simulink model "simulacaoPI"  (R2023b)
settings: Solver=VariableStepAuto  StartTime=0.0  StopTime=0.05  RelTol=1e-3
values from neighbouring files (symbols this model uses):
  Cc = 0.000143    [PI_boost.m]
  Ts = 5.0e-5    (= 5e-05)    [PI_boost.m]
  Vs = 30    [PI_boost.m]
libraries: spsSeriesRLCBranchLib x3, spsCurrentMeasurementLib x1, spsDiodeLib x1, spsDCVoltageSourceLib x1, spsGroundLib x1, spsMosfetLib x1, spsPWMGeneratorDCDCLib x1, spsVoltageMeasurementLib x1, sps_lib x1
settings Model: Creator=luisf  LastModifiedBy=luisf

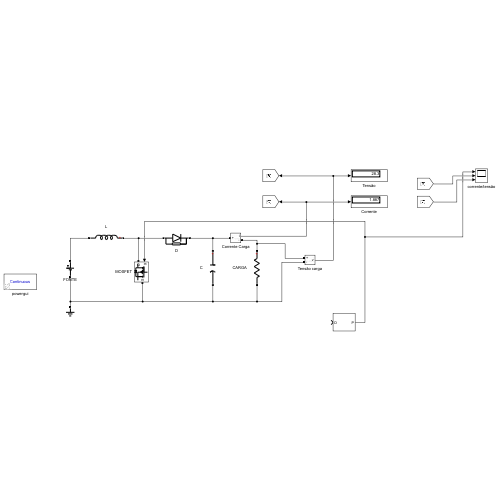
[thumbnail: Simulink's stored preview of the top-level diagram]
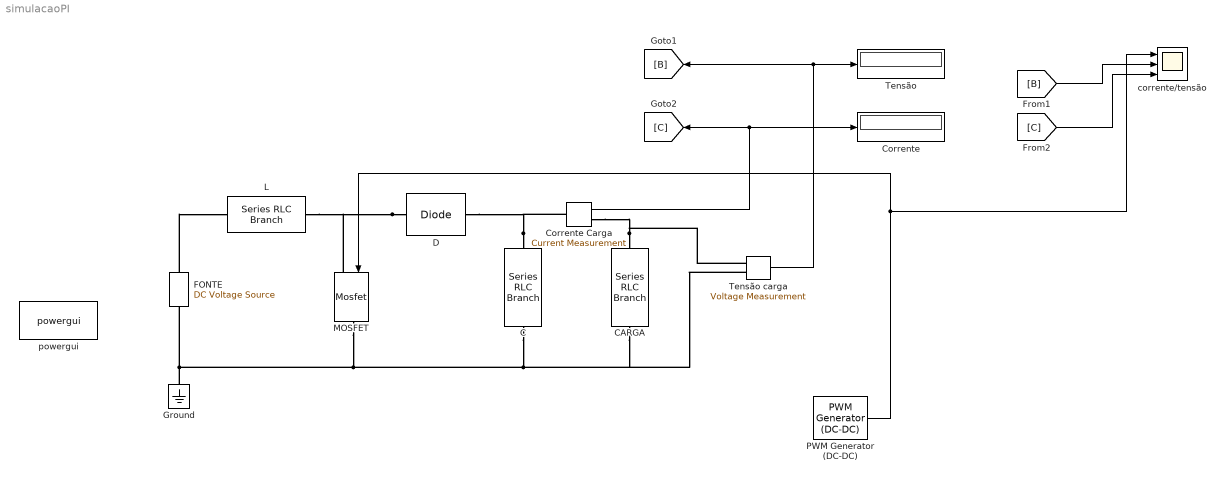
== system simulacaoPI ==
  C : spsSeriesRLCBranchLib/Series RLC Branch  LConnTagsString=__new0  RConnTagsString=__new0  BranchType=C  Resistance=1  Inductance=1e-3  SetiL0=off  InitialCurrent=0  Capacitance=Cc  Setx0=off  InitialVoltage=0  Measurements=None
  CARGA : spsSeriesRLCBranchLib/Series RLC Branch  LConnTagsString=__new0  RConnTagsString=__new0  BranchType=R  Resistance=15  Inductance=1e-3  SetiL0=off  InitialCurrent=0  Capacitance=1e-6  Setx0=off  InitialVoltage=0  Measurements=None
  Corrente : Display
  Corrente Carga : spsCurrentMeasurementLib/Current Measurement  PhasorSimulation=off  OutputType=Complex  PSBequivalent=0
  D : spsDiodeLib/Diode  Ron=0.001  Lon=0  Vf=1.7  IC=0  UseSnubber=0  Rs=500  Cs=250e-9  Measurements=off
  FONTE : spsDCVoltageSourceLib/DC Voltage Source  Amplitude=Vs  Measurements=None
  Ground : spsGroundLib/Ground  LConnTagsString=a
  L : spsSeriesRLCBranchLib/Series RLC Branch  LConnTagsString=__new0  RConnTagsString=__new0  BranchType=L  Resistance=1  Inductance=0.00056  SetiL0=off  InitialCurrent=0  Capacitance=1e-6  Setx0=off  InitialVoltage=0  Measurements=None
  MOSFET : spsMosfetLib/Mosfet  Ron=0.1  Lon=0  Rd=0.01  Vfd=0  IC=0  Rs=1e5  Cs=inf  Measurements=off
  PWM Generator (DC-DC) : spsPWMGeneratorDCDCLib/PWM Generator (DC-DC)  Fsw=20000  Ts=1/Ts
  Tensão : Display
  Tensão carga : spsVoltageMeasurementLib/Voltage Measurement  PhasorSimulation=off  OutputType=Complex  PSBequivalent=0
  corrente/tensão : Scope  NumInputPorts=3
  powergui : sps_lib/powergui  Priority=1  SimulationMode=Continuous  SampleTime=50e-6  frequency=60  Iterations=50  frequencyindice=0  Pbase=100e6  ErrMax=1e-4  UnitsV=kV  UnitsW=MW  buscounter=0  FunctionMessages=off  echomessages=off  EnableUseOfTLC=off  CurrentSourceSwitches=off  DisableSnubberDevices=off  DisableRonSwitches=off  DisableVfSwitches=off  DisplayEquations=off  AutomaticDiscreteSolvers=off  SolverType=Tustin/Backward Euler (TBE)  Interpol=off  ExternalGateDelay=off  methode=off  Ts=100  x0status=blocks  SPID=on  SwTol=0  HookPort=off  NonlinearTolerance=1e-4  nMaxIteration=100  ContinueOnMaxIteration=off  RestoreLinks=warning  ResistiveCurrentMeasurement=off  Frange=[0:2:500]  Ylog=off  Xlog=on  ShowGrid=off  save=off  variable=ZData  structure=0  ZoomFFT=off  StartTime=0.0  cycles=1  DisplayStyle=1  fundamental=60  FreqAxis=off  MaxFrequency=1000  frequencyindicesteady=1  RmsSteady=1  display=off
  wires:
  [B] -> corrente/tensão/2
  Corrente Carga/1 -> [C], Corrente/1
  [C] -> corrente/tensão/3
  Tensão carga/1 -> Tensão/1, [B]
  PWM Generator (DC-DC)/1 -> corrente/tensão/1, MOSFET/1
  connections:
  D/LConn1 -- L/LConn1 -- MOSFET/LConn1
  C/RConn1 -- Ground/LConn1 -- FONTE/LConn1 -- MOSFET/RConn1 -- Tensão carga/LConn2 -- CARGA/RConn1
  CARGA/LConn1 -- Corrente Carga/RConn1 -- Tensão carga/LConn1
  C/LConn1 -- D/RConn1 -- Corrente Carga/LConn1
  FONTE/RConn1 -- L/RConn1
